simulink model "H05_ERR_Szinusz"  (R2026a)
settings: Solver=VariableStepAuto  MaxStep=tau/25
InitFcn:
  | tau = 1;
libraries: MK_H x2, simulink_extras x1
settings Model: Creator=Szalay  LastModifiedBy=Szalay

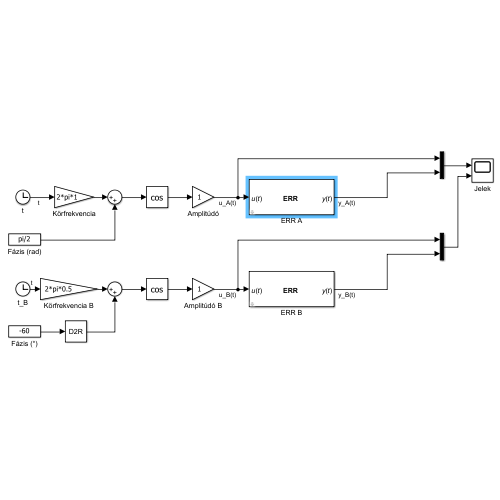
[thumbnail: Simulink's stored preview of the top-level diagram]
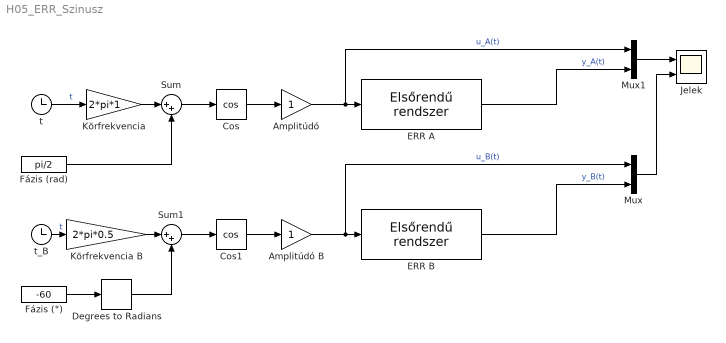
== system H05_ERR_Szinusz ==
  Amplitúdó : Gain
  Amplitúdó B : Gain
  Cos : Trigonometry  Operator=cos
  Cos1 : Trigonometry  Operator=cos
  Degrees to Radians : simulink_extras/Transformations/Degrees to Radians
  ERR A : MK_H/Elsőrendű rendszer  K=1  tau=tau  y_0=0
  ERR B : MK_H/Elsőrendű rendszer  K=1  tau=tau  y_0=0
  Fázis (rad) : Constant  Value=pi/2
  Fázis (°) : Constant  Value=-60
  Jelek : Scope  NumInputPorts=2
      settings: ActiveDisplayYMinimum=-0.39110281891080279  ActiveDisplayYMaximum=0.48312701159569782
  Körfrekvencia : Gain  Gain=2*pi*1
  Körfrekvencia B : Gain  Gain=2*pi*0.5
  Mux : Mux  Inputs=2
  Mux1 : Mux  Inputs=2
  Sum : Sum  Inputs=|++
  Sum1 : Sum  Inputs=|++
  t : Clock
  t_B : Clock
  wires:
  Mux/1 -> Jelek/2
  ERR A/1 -> Mux1/2  "y_A(t)"
  ERR B/1 -> Mux/2  "y_B(t)"
  t/1 -> Körfrekvencia/1  "t"
  Körfrekvencia/1 -> Sum/1
  Sum/1 -> Cos/1
  Cos/1 -> Amplitúdó/1
  Amplitúdó/1 -> Mux1/1, ERR A/1  "u_A(t)"
  Fázis (rad)/1 -> Sum/2
  Mux1/1 -> Jelek/1
  Fázis (°)/1 -> Degrees to Radians/1
  Amplitúdó B/1 -> Mux/1, ERR B/1  "u_B(t)"
  Cos1/1 -> Amplitúdó B/1
  Sum1/1 -> Cos1/1
  Körfrekvencia B/1 -> Sum1/1
  t_B/1 -> Körfrekvencia B/1  "t"
  Degrees to Radians/1 -> Sum1/2
